simulink model "Motor_model_with_controller_sampling"  (R2026a)
settings: Solver=VariableStepAuto  StopTime=0.6
values from neighbouring files (symbols this model uses):
  D = 3.2e-7    (= 3.2e-07)    [script_simulink_sampling_effect.m]
  gear = 9.68    [MATLAB_script_data_sampling_effect.m]    (also in script_simulink_sampling_effect.m = 9.6)
  J_new = 5.4836e-6    (= 5.4836e-06)    [script_simulink_sampling_effect.m]
  Kb = 0.009    [script_simulink_sampling_effect.m]
  Kp_P = 0.05    [script_simulink_sampling_effect.m]
  Kt = 0.009    [script_simulink_sampling_effect.m]
  L = 0.01    [script_simulink_sampling_effect.m]
  R = 6.8    [script_simulink_sampling_effect.m]
  Ts = 0.001    [script_simulink_sampling_effect.m]
  wrad = 0.03    [MATLAB_script_data_sampling_effect.m]    (also in script_simulink_sampling_effect.m = 0.0315)
settings Model: Creator=sahra  LastModifiedBy=sahra

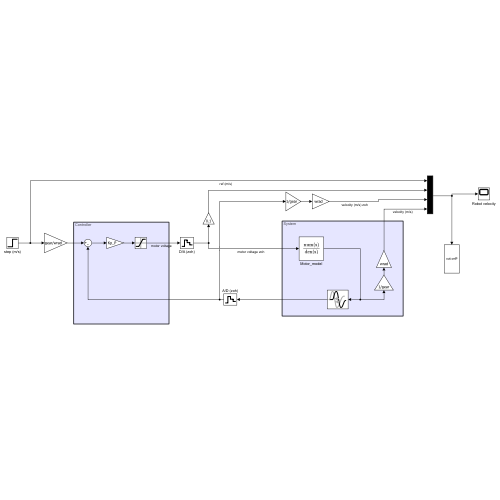
[thumbnail: Simulink's stored preview of the top-level diagram]
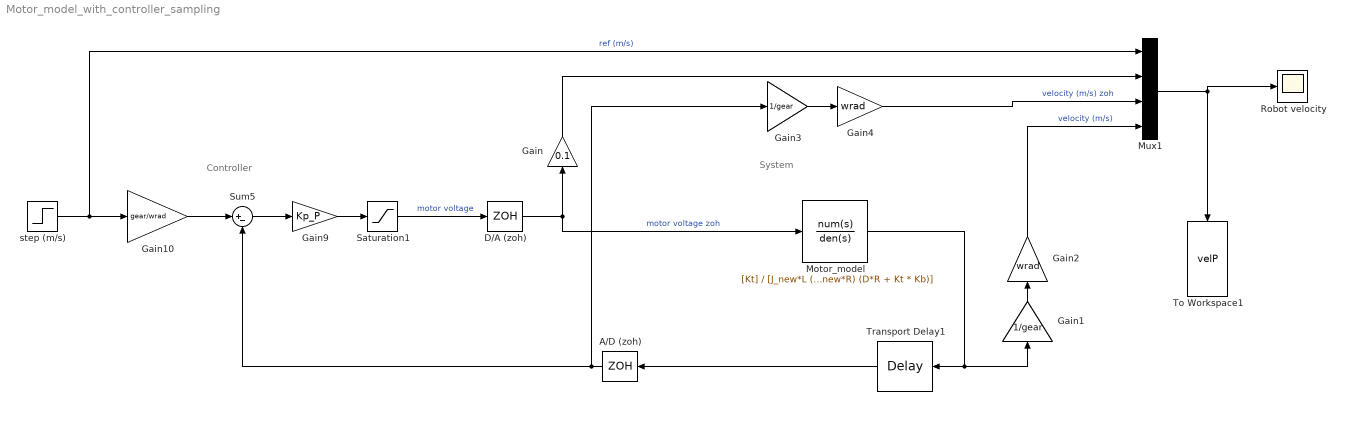
== system Motor_model_with_controller_sampling ==
  note: Controller
  note: System
  A/D (zoh) : ZeroOrderHold  SampleTime=Ts
  D/A (zoh) : ZeroOrderHold  SampleTime=Ts
  Gain : Gain  Gain=0.1
  Gain1 : Gain  Gain=1/gear
  Gain10 : Gain  Gain=gear/wrad
  Gain2 : Gain  Gain=wrad
  Gain3 : Gain  Gain=1/gear
  Gain4 : Gain  Gain=wrad
  Gain9 : Gain  Gain=Kp_P
  Motor_model : TransferFcn  Numerator=[Kt]  Denominator=[J_new*L (D*L + J_new*R) (D*R + Kt * Kb)]
  Mux1 : Mux
  Robot velocity : Scope
      settings: ActiveDisplayYMinimum=-60.754208750467939  ActiveDisplayYMaximum=134.00460786451399
  Saturation1 : Saturate  UpperLimit=9  LowerLimit=-9
  Sum5 : Sum  Inputs=|+-
  To Workspace1 : ToWorkspace  VariableName=velP  SaveFormat=Timeseries  SampleTime=-1
  Transport Delay1 : TransportDelay  DelayTime=0.01
  step (m/s) : Step  Time=0.1  FinalValue=0.1  SampleTime=0
  wires:
  Gain10/1 -> Sum5/1
  step (m/s)/1 -> Gain10/1, Mux1/1  "ref (m/s)"
  Gain9/1 -> Saturation1/1
  Sum5/1 -> Gain9/1
  Saturation1/1 -> D/A (zoh)/1  "motor voltage"
  Mux1/1 -> Robot velocity/1, To Workspace1/1
  D/A (zoh)/1 -> Motor_model/1, Gain/1  "motor voltage zoh"
  Gain/1 -> Mux1/2
  Motor_model/1 -> Gain1/1, Transport Delay1/1
  Gain1/1 -> Gain2/1
  Gain2/1 -> Mux1/4  "velocity (m/s)"
  Transport Delay1/1 -> A/D (zoh)/1
  A/D (zoh)/1 -> Sum5/2, Gain3/1
  Gain3/1 -> Gain4/1
  Gain4/1 -> Mux1/3  "velocity (m/s) zoh"
